simulink model "harness"  (R2026a)
settings: Solver=ode4  FixedStep=0.001
settings Model: Creator=muthi  LastModifiedBy=muthi

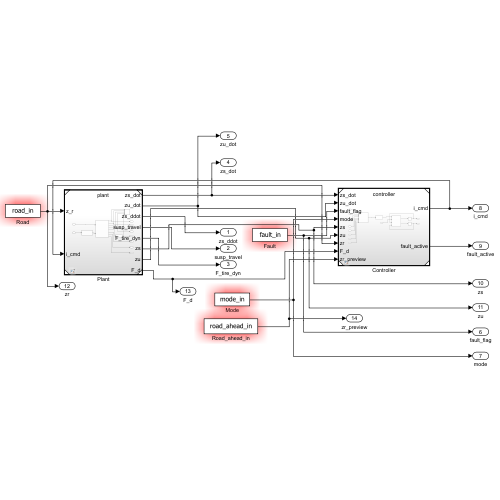
[thumbnail: Simulink's stored preview of the top-level diagram]
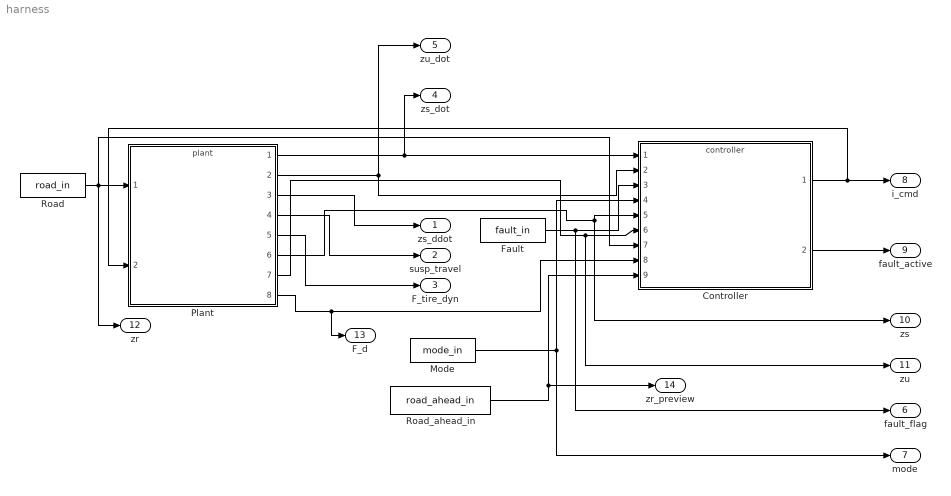
== system harness ==
  Controller : ModelReference  ModelNameDialog=controller  SimulationMode=Normal  ModelReferenceVersion=1.23
  Fault : FromWorkspace  VariableName=fault_in  SampleTime=0.001  Interpolate=off  OutputAfterFinalValue=Holding final value
  Mode : FromWorkspace  VariableName=mode_in  SampleTime=0.001  Interpolate=off  OutputAfterFinalValue=Holding final value
  Plant : ModelReference  ModelNameDialog=plant  SimulationMode=Normal  ModelReferenceVersion=1.9
  Road : FromWorkspace  VariableName=road_in  OutputAfterFinalValue=Holding final value
  Road_ahead_in : FromWorkspace  VariableName=road_ahead_in  OutputAfterFinalValue=Holding final value
  zs_ddot : Outport
  susp_travel : Outport  Port=2
  F_tire_dyn : Outport  Port=3
  zs_dot : Outport  Port=4
  zu_dot : Outport  Port=5
  fault_flag : Outport  Port=6
  mode : Outport  Port=7
  i_cmd : Outport  Port=8
  fault_active : Outport  Port=9
  zs : Outport  Port=10
  zu : Outport  Port=11
  zr : Outport  Port=12
  F_d : Outport  Port=13
  zr_preview : Outport  Port=14
  wires:
  Road/1 -> zr/1, Controller/7, Plant/1
  Controller/1 -> i_cmd/1, Plant/2
  Plant/1 -> Controller/1, zs_dot/1
  Plant/2 -> Controller/2, zu_dot/1
  Mode/1 -> Controller/4, mode/1
  Plant/4 -> susp_travel/1
  Plant/5 -> F_tire_dyn/1
  Plant/3 -> zs_ddot/1
  Controller/2 -> fault_active/1
  Plant/8 -> F_d/1, Controller/8
  Plant/6 -> zs/1, Controller/5
  Plant/7 -> zu/1, Controller/6
  Fault/1 -> fault_flag/1, Controller/3
  Road_ahead_in/1 -> zr_preview/1, Controller/9
